simulink model "NBMS_App_Harness1"  (R2026b)
settings: Solver=FixedStepDiscrete  StopTime=25  FixedStep=0.1
undefined symbols (not defined in the file): Active_DisChrg_E, BMS_BattSoCDerate_E, BMS_BattTempDerate_E, BMS_DCDCMosfet_STS_E, BMS_HVMosfet_STS_E, BMS_MODE_E, BMS_NM_Msg_E, BMS_PMosfet_STS_E, Charger_Mode_E, Charger_Mode_Req_E, CV_Mode_Timer_E, OBC_E, VDU_MACHINE_STS_E
(part 1 of 4)
settings Model: PauseTimes=12  Creator=rathi  LastModifiedBy=rathi
settings OptimizationCC: DefaultParameterBehavior=Inlined  DifferentSizesBufferReuse=on  EfficientTunableParamExpr=on  EnhancedBackFolding=on  OptimizationCustomize=off  OptimizeBlockOrder=speed  PassReuseOutputArgsAs=Individual arguments  RemoveInternalMemoryZeroInit=on  RemoveRootLevelIOMemoryZeroInit=on
settings DebuggingCC: ParameterTunabilityLossMsg=error
settings SFSimCC: MATLABDynamicMemAlloc=off
settings RTWCC: Description=Embedded Coder  GenCodeOnly=on  PackageGeneratedCodeAndArtifacts=on  SystemTargetFile=ert.tlc  TemplateMakefile=ert_default_tmf
settings CodeAppCC: ForceParamTrailComments=on  IgnoreCustomStorageClasses=off  InsertBlockDesc=on  OperatorAnnotations=on  SFDataObjDesc=on  SimulinkDataObjDesc=on
settings ERTTargetCC: DynamicArrayContainerType=coder::array  GenerateSampleERTMain=on
settings ConfigComp: DVDefectChecker=on  DVDetectOutOfBounds=on  DVHarnessSource=Signal Editor  DVModelReferenceHarness=on  DVTestSuiteOptimization=Auto

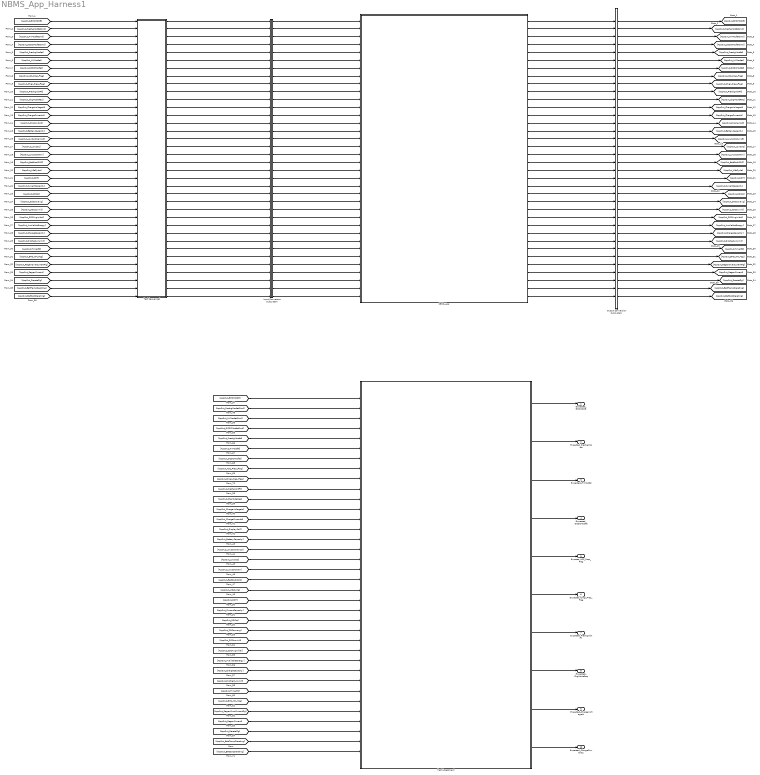
== system NBMS_App_Harness1 ==
  Input Conversion Subsystem : Subsystem  Tag=__SLT_ICS__  Description=|
      | Signal spec.
      | and routing
      settings: AttributesFormatString=%<Description>
  NBMS_App : ModelReference  ModelNameDialog=NBMS_App  SimulationMode=Normal  ModelReferenceVersion=1.0
  Output Conversion Subsystem : Subsystem  Tag=__SLT_OCS__  Description=|
      | Signal spec.
      | and routing
      settings: AttributesFormatString=%<Description>
  Test Assessment : Test Sequence  TreatAsAtomicUnit=on
  Test Sequence1 : Test Sequence  TreatAsAtomicUnit=on
  Expected_BMSMODE : Outport
  Expected_PrechgMosfet : Outport  Port=2
  Expected_HVMosfet : Outport  Port=3
  Expected_DCDCMosfet : Outport  Port=4
  Expcted_ASC_Prep_Flag : Outport  Port=5
  Expected_Chrgr_Prep_Flag : Outport  Port=6
  Expected_PrechgVoltFlt : Outport  Port=7
  Expected_ChgModeReq : Outport  Port=8
  Expected_ChargeVoltageLt : Outport  Port=9
  Expected_ChargeCurrentLt : Outport  Port=10
  wires:
  Test Sequence1/1(AppIn_HardwiredIgn) -> Input Conversion Subsystem/1(Inport_1)
  Test Sequence1/2(AppIn_OBCwakeup) -> Input Conversion Subsystem/2(Inport_2)
  Test Sequence1/3(AppIn_RTCwakeup) -> Input Conversion Subsystem/3(Inport_3)
  Test Sequence1/4(AppIn_MCUHVIL) -> Input Conversion Subsystem/4(Inport_4)
  Test Sequence1/5(AppIn_OBCHVIL) -> Input Conversion Subsystem/5(Inport_5)
  Test Sequence1/6(AppIn_SoCLEDSW) -> Input Conversion Subsystem/6(Inport_6)
  Test Sequence1/7(AppIn_ChgMode) -> Input Conversion Subsystem/7(Inport_7)
  Test Sequence1/8(AppIn_CVmodeTimer) -> Input Conversion Subsystem/8(Inport_8)
  Test Sequence1/9(AppIn_TRerror) -> Input Conversion Subsystem/9(Inport_9)
  Test Sequence1/10(AppIn_TRtimer) -> Input Conversion Subsystem/10(Inport_10)
  Test Sequence1/11(AppIn_G3CommonFlt) -> Input Conversion Subsystem/11(Inport_11)
  Test Sequence1/12(AppIn_G3DischargeFlt) -> Input Conversion Subsystem/12(Inport_12)
  Test Sequence1/13(AppIn_G4T1DischargeFlt) -> Input Conversion Subsystem/13(Inport_13)
  Test Sequence1/14(AppIn_G4T2DischargeFlt) -> Input Conversion Subsystem/14(Inport_14)
  Test Sequence1/15(AppIn_G4CommonFlt) -> Input Conversion Subsystem/15(Inport_15)
  Test Sequence1/16(AppIn_G4ChargeFlt) -> Input Conversion Subsystem/16(Inport_16)
  Test Sequence1/17(AppIn_OBCHeartbeatFail) -> Input Conversion Subsystem/17(Inport_17)
  Test Sequence1/18(AppIn_LoadVolt) -> Input Conversion Subsystem/18(Inport_18)
  Test Sequence1/19(AppIn_PackVolt) -> Input Conversion Subsystem/19(Inport_19)
  Test Sequence1/20(AppIn_ActiveDischg) -> Input Conversion Subsystem/20(Inport_20)
  Test Sequence1/21(AppIn_BattTemp) -> Input Conversion Subsystem/21(Inport_21)
  Test Sequence1/22(AppIn_BattCurrent) -> Input Conversion Subsystem/22(Inport_22)
  Test Sequence1/23(AppIn_BattVoltages) -> Input Conversion Subsystem/23(Inport_23)
  Test Sequence1/24(AppIn_LastStoredSOC) -> Input Conversion Subsystem/24(Inport_24)
  Test Sequence1/25(AppIn_LastStoredCycle) -> Input Conversion Subsystem/25(Inport_25)
  Test Sequence1/26(AppIn_I2Cerror) -> Input Conversion Subsystem/26(Inport_26)
  Test Sequence1/27(AppIn_LastStoredSOH) -> Input Conversion Subsystem/27(Inport_27)
  Test Sequence1/28(AppIn_MachineStatus) -> Input Conversion Subsystem/28(Inport_28)
  Test Sequence1/29(AppIn_HVMosfetfb) -> Input Conversion Subsystem/29(Inport_29)
  Test Sequence1/30(AppIn_DCDCMosfetfb) -> Input Conversion Subsystem/30(Inport_30)
  Test Sequence1/31(AppIn_PMosfetfb) -> Input Conversion Subsystem/31(Inport_31)
  Test Sequence1/32(AppIn_BMSVltSnsrFail) -> Input Conversion Subsystem/32(Inport_32)
  Test Sequence1/33(AppIn_BattPackTempSnsrFail) -> Input Conversion Subsystem/33(Inport_33)
  Test Sequence1/34(AppIn_VltImbFlt) -> Input Conversion Subsystem/34(Inport_34)
  Test Sequence1/35(AppIn_TempImbWarn) -> Input Conversion Subsystem/35(Inport_35)
  Test Sequence1/36(AppIn_EEPROMSoCWarn15) -> Input Conversion Subsystem/36(Inport_36)
  [AppOut_BMSMODE] -> Test Sequence1/1(AppOut_BMSMODE)
  [AppOut_PrechgMosfetCmd] -> Test Sequence1/2(AppOut_PrechgMosfetCmd)
  [AppOut_HVMosfetCmd] -> Test Sequence1/3(AppOut_HVMosfetCmd)
  [AppOut_DCDCMosfetCmd] -> Test Sequence1/4(AppOut_DCDCMosfetCmd)
  [AppOut_PrechgMosfet] -> Test Sequence1/5(AppOut_PrechgMosfet)
  [AppOut_HVMosfet] -> Test Sequence1/6(AppOut_HVMosfet)
  [AppOut_DCDCMosfet] -> Test Sequence1/7(AppOut_DCDCMosfet)
  [AppOut_ASC_Prep_Flag] -> Test Sequence1/8(AppOut_ASC_Prep_Flag)
  [AppOut_Chrgr_Prep_Flag] -> Test Sequence1/9(AppOut_Chrgr_Prep_Flag)
  [AppOut_PrechgVoltFlt] -> Test Sequence1/10(AppOut_PrechgVoltFlt)
  [AppOut_ChgModeReq] -> Test Sequence1/11(AppOut_ChgModeReq)
  [AppOut_ChargeVoltageLt] -> Test Sequence1/12(AppOut_ChargeVoltageLt)
  [AppOut_ChargeCurrentLt] -> Test Sequence1/13(AppOut_ChargeCurrentLt)
  [AppOut_DisplaySoC] -> Test Sequence1/14(AppOut_DisplaySoC)
  [AppOut_BatteryCapacity] -> Test Sequence1/15(AppOut_BatteryCapacity)
  [AppOut_LowSoCWarn15] -> Test Sequence1/16(AppOut_LowSoCWarn15)
  [AppOut_LowSoC] -> Test Sequence1/17(AppOut_LowSoC)
  [AppOut_LowSoCWarn] -> Test Sequence1/18(AppOut_LowSoCWarn)
  [AppOut_BattPackSOC] -> Test Sequence1/19(AppOut_BattPackSOC)
  [AppOut_LifeCycle] -> Test Sequence1/20(AppOut_LifeCycle)
  [AppOut_SOH] -> Test Sequence1/21(AppOut_SOH)
  [AppOut_CurrentCapacity] -> Test Sequence1/22(AppOut_CurrentCapacity)
  [AppOut_SOCcc] -> Test Sequence1/23(AppOut_SOCcc)
  [AppOut_SOCocvavg] -> Test Sequence1/24(AppOut_SOCocvavg)
  [AppOut_SOCocvInit] -> Test Sequence1/25(AppOut_SOCocvInit)
  [AppOut_SOCAvgInitial] -> Test Sequence1/26(AppOut_SOCAvgInitial)
  [AppOut_AvailableEnergy] -> Test Sequence1/27(AppOut_AvailableEnergy)
  [AppOut_ChargeCapacity] -> Test Sequence1/28(AppOut_ChargeCapacity)
  [AppOut_DischgCurrLimit] -> Test Sequence1/29(AppOut_DischgCurrLimit)
  [AppOut_Timer30] -> Test Sequence1/30(AppOut_Timer30)
  [AppOut_BMS_NM_Msg] -> Test Sequence1/31(AppOut_BMS_NM_Msg)
  [AppOut_RegenOverCurrentFlg] -> Test Sequence1/32(AppOut_RegenOverCurrentFlg)
  [AppOut_RegenCurrent] -> Test Sequence1/33(AppOut_RegenCurrent)
  [AppOut_DerateFlg] -> Test Sequence1/34(AppOut_DerateFlg)
  [AppOut_BattTempDerating] -> Test Sequence1/35(AppOut_BattTempDerating)
  [AppOut_BattSoCDerating] -> Test Sequence1/36(AppOut_BattSoCDerating)
  Output Conversion Subsystem/1(Outport_1) -> [AppOut_BMSMODE]  "AppOut_BMSMODE"
  Output Conversion Subsystem/2(Outport_2) -> [AppOut_PrechgMosfetCmd]  "AppOut_PrechgMosfetCmd"
  Output Conversion Subsystem/3(Outport_3) -> [AppOut_HVMosfetCmd]  "AppOut_HVMosfetCmd"
  Output Conversion Subsystem/4(Outport_4) -> [AppOut_DCDCMosfetCmd]  "AppOut_DCDCMosfetCmd"
  Output Conversion Subsystem/5(Outport_5) -> [AppOut_PrechgMosfet]  "AppOut_PrechgMosfet"
  Output Conversion Subsystem/6(Outport_6) -> [AppOut_HVMosfet]  "AppOut_HVMosfet"
  Output Conversion Subsystem/7(Outport_7) -> [AppOut_DCDCMosfet]  "AppOut_DCDCMosfet"
  Output Conversion Subsystem/8(Outport_8) -> [AppOut_ASC_Prep_Flag]  "AppOut_ASC_Prep_Flag"
  Output Conversion Subsystem/9(Outport_9) -> [AppOut_Chrgr_Prep_Flag]  "AppOut_Chrgr_Prep_Flag"
  Output Conversion Subsystem/10(Outport_10) -> [AppOut_PrechgVoltFlt]  "AppOut_PrechgVoltFlt"
  Output Conversion Subsystem/11(Outport_11) -> [AppOut_ChgModeReq]  "AppOut_ChgModeReq"
  Output Conversion Subsystem/12(Outport_12) -> [AppOut_ChargeVoltageLt]  "AppOut_ChargeVoltageLt"
  Output Conversion Subsystem/13(Outport_13) -> [AppOut_ChargeCurrentLt]  "AppOut_ChargeCurrentLt"
  Output Conversion Subsystem/14(Outport_14) -> [AppOut_DisplaySoC]  "AppOut_DisplaySoC"
  Output Conversion Subsystem/15(Outport_15) -> [AppOut_BatteryCapacity]  "AppOut_BatteryCapacity"
  Output Conversion Subsystem/16(Outport_16) -> [AppOut_LowSoCWarn15]  "AppOut_LowSoCWarn15"
  Output Conversion Subsystem/17(Outport_17) -> [AppOut_LowSoC]  "AppOut_LowSoC"
  Output Conversion Subsystem/18(Outport_18) -> [AppOut_LowSoCWarn]  "AppOut_LowSoCWarn"
  Output Conversion Subsystem/19(Outport_19) -> [AppOut_BattPackSOC]  "AppOut_BattPackSOC"
  Output Conversion Subsystem/20(Outport_20) -> [AppOut_LifeCycle]  "AppOut_LifeCycle"
  Output Conversion Subsystem/21(Outport_21) -> [AppOut_SOH]  "AppOut_SOH"
  Output Conversion Subsystem/22(Outport_22) -> [AppOut_CurrentCapacity]  "AppOut_CurrentCapacity"
  Output Conversion Subsystem/23(Outport_23) -> [AppOut_SOCcc]  "AppOut_SOCcc"
  Output Conversion Subsystem/24(Outport_24) -> [AppOut_SOCocvavg]  "AppOut_SOCocvavg"
  Output Conversion Subsystem/25(Outport_25) -> [AppOut_SOCocvInit]  "AppOut_SOCocvInit"
  Output Conversion Subsystem/26(Outport_26) -> [AppOut_SOCAvgInitial]  "AppOut_SOCAvgInitial"
  Output Conversion Subsystem/27(Outport_27) -> [AppOut_AvailableEnergy]  "AppOut_AvailableEnergy"
  Output Conversion Subsystem/28(Outport_28) -> [AppOut_ChargeCapacity]  "AppOut_ChargeCapacity"
  Output Conversion Subsystem/29(Outport_29) -> [AppOut_DischgCurrLimit]  "AppOut_DischgCurrLimit"
  Output Conversion Subsystem/30(Outport_30) -> [AppOut_Timer30]  "AppOut_Timer30"
  Output Conversion Subsystem/31(Outport_31) -> [AppOut_BMS_NM_Msg]  "AppOut_BMS_NM_Msg"
  Output Conversion Subsystem/32(Outport_32) -> [AppOut_RegenOverCurrentFlg]  "AppOut_RegenOverCurrentFlg"
  Output Conversion Subsystem/33(Outport_33) -> [AppOut_RegenCurrent]  "AppOut_RegenCurrent"
  Output Conversion Subsystem/34(Outport_34) -> [AppOut_DerateFlg]  "AppOut_DerateFlg"
  Output Conversion Subsystem/35(Outport_35) -> [AppOut_BattTempDerating]  "AppOut_BattTempDerating"
  Output Conversion Subsystem/36(Outport_36) -> [AppOut_BattSoCDerating]  "AppOut_BattSoCDerating"
  [AppOut_Chrgr_Prep_Flag] -> Test Assessment/9(AppOut_Chrgr_Prep_Flag)
  [AppOut_BattSoCDerating] -> Test Assessment/36(AppOut_BattSoCDerating)
  Test Assessment/1(Expected_BMSMODE) -> Expected_BMSMODE/1
  [AppOut_PrechgMosfet] -> Test Assessment/5(AppOut_PrechgMosfet)
  [AppOut_ChargeCapacity] -> Test Assessment/28(AppOut_ChargeCapacity)
  [AppOut_DerateFlg] -> Test Assessment/34(AppOut_DerateFlg)
  [AppOut_BMSMODE] -> Test Assessment/1(AppOut_BMSMODE)
  [AppOut_LowSoCWarn15] -> Test Assessment/16(AppOut_LowSoCWarn15)
  [AppOut_SOCocvInit] -> Test Assessment/25(AppOut_SOCocvInit)
  [AppOut_HVMosfet] -> Test Assessment/6(AppOut_HVMosfet)
  [AppOut_DisplaySoC] -> Test Assessment/14(AppOut_DisplaySoC)
  [AppOut_DischgCurrLimit] -> Test Assessment/29(AppOut_DischgCurrLimit)
  [AppOut_Timer30] -> Test Assessment/30(AppOut_Timer30)
  Test Assessment/4(Expected_DCDCMosfet) -> Expected_DCDCMosfet/1
  [AppOut_BatteryCapacity] -> Test Assessment/15(AppOut_BatteryCapacity)
  Test Assessment/7(Expected_PrechgVoltFlt) -> Expected_PrechgVoltFlt/1
  [AppOut_BMS_NM_Msg] -> Test Assessment/31(AppOut_BMS_NM_Msg)
  [AppOut_SOCAvgInitial] -> Test Assessment/26(AppOut_SOCAvgInitial)
  [AppOut_RegenOverCurrentFlg] -> Test Assessment/32(AppOut_RegenOverCurrentFlg)
  Test Assessment/6(Expected_Chrgr_Prep_Flag) -> Expected_Chrgr_Prep_Flag/1
  [AppOut_LifeCycle] -> Test Assessment/20(AppOut_LifeCycle)
  [AppOut_RegenCurrent] -> Test Assessment/33(AppOut_RegenCurrent)
  [AppOut_HVMosfetCmd] -> Test Assessment/3(AppOut_HVMosfetCmd)
  [AppOut_PrechgMosfetCmd] -> Test Assessment/2(AppOut_PrechgMosfetCmd)
  [AppOut_BattTempDerating] -> Test Assessment/35(AppOut_BattTempDerating)
  [AppOut_PrechgVoltFlt] -> Test Assessment/10(AppOut_PrechgVoltFlt)
  [AppOut_SOH] -> Test Assessment/21(AppOut_SOH)
  [AppOut_ChargeVoltageLt] -> Test Assessment/12(AppOut_ChargeVoltageLt)
  [AppOut_LowSoCWarn] -> Test Assessment/18(AppOut_LowSoCWarn)
  Test Assessment/3(Expected_HVMosfet) -> Expected_HVMosfet/1
  [AppOut_ASC_Prep_Flag] -> Test Assessment/8(AppOut_ASC_Prep_Flag)
  [AppOut_CurrentCapacity] -> Test Assessment/22(AppOut_CurrentCapacity)
  [AppOut_AvailableEnergy] -> Test Assessment/27(AppOut_AvailableEnergy)
  Test Assessment/5(Expected_ASC_Prep_Flag) -> Expcted_ASC_Prep_Flag/1
  [AppOut_ChgModeReq] -> Test Assessment/11(AppOut_ChgModeReq)
  [AppOut_SOCcc] -> Test Assessment/23(AppOut_SOCcc)
  Test Assessment/2(Expected_PrechgMosfet) -> Expected_PrechgMosfet/1
  [AppOut_BattPackSOC] -> Test Assessment/19(AppOut_BattPackSOC)
  [AppOut_DCDCMosfet] -> Test Assessment/7(AppOut_DCDCMosfet)
  [AppOut_LowSoC] -> Test Assessment/17(AppOut_LowSoC)
  [AppOut_DCDCMosfetCmd] -> Test Assessment/4(AppOut_DCDCMosfetCmd)
  [AppOut_SOCocvavg] -> Test Assessment/24(AppOut_SOCocvavg)
  [AppOut_ChargeCurrentLt] -> Test Assessment/13(AppOut_ChargeCurrentLt)
  Test Assessment/8(Expected_ChgModeReq) -> Expected_ChgModeReq/1
  Test Assessment/9(Expected_ChargeVoltageLt) -> Expected_ChargeVoltageLt/1
  Test Assessment/10(Expected_ChargeCurrentLt) -> Expected_ChargeCurrentLt/1
  NBMS_App/1 -> Output Conversion Subsystem/1(Inport_1)
  NBMS_App/2 -> Output Conversion Subsystem/2(Inport_2)
  NBMS_App/3 -> Output Conversion Subsystem/3(Inport_3)
  NBMS_App/4 -> Output Conversion Subsystem/4(Inport_4)
  NBMS_App/5 -> Output Conversion Subsystem/5(Inport_5)
  NBMS_App/6 -> Output Conversion Subsystem/6(Inport_6)
  NBMS_App/7 -> Output Conversion Subsystem/7(Inport_7)
  NBMS_App/8 -> Output Conversion Subsystem/8(Inport_8)
  NBMS_App/9 -> Output Conversion Subsystem/9(Inport_9)
  NBMS_App/10 -> Output Conversion Subsystem/10(Inport_10)
  NBMS_App/11 -> Output Conversion Subsystem/11(Inport_11)
  NBMS_App/12 -> Output Conversion Subsystem/12(Inport_12)
  NBMS_App/13 -> Output Conversion Subsystem/13(Inport_13)
  NBMS_App/14 -> Output Conversion Subsystem/14(Inport_14)
  NBMS_App/15 -> Output Conversion Subsystem/15(Inport_15)
  NBMS_App/16 -> Output Conversion Subsystem/16(Inport_16)
  NBMS_App/17 -> Output Conversion Subsystem/17(Inport_17)
  NBMS_App/18 -> Output Conversion Subsystem/18(Inport_18)
  NBMS_App/19 -> Output Conversion Subsystem/19(Inport_19)
  NBMS_App/20 -> Output Conversion Subsystem/20(Inport_20)
  NBMS_App/21 -> Output Conversion Subsystem/21(Inport_21)
  NBMS_App/22 -> Output Conversion Subsystem/22(Inport_22)
  NBMS_App/23 -> Output Conversion Subsystem/23(Inport_23)
  NBMS_App/24 -> Output Conversion Subsystem/24(Inport_24)
  NBMS_App/25 -> Output Conversion Subsystem/25(Inport_25)
  NBMS_App/26 -> Output Conversion Subsystem/26(Inport_26)
  NBMS_App/27 -> Output Conversion Subsystem/27(Inport_27)
  NBMS_App/28 -> Output Conversion Subsystem/28(Inport_28)
  NBMS_App/29 -> Output Conversion Subsystem/29(Inport_29)
  NBMS_App/30 -> Output Conversion Subsystem/30(Inport_30)
  NBMS_App/31 -> Output Conversion Subsystem/31(Inport_31)
  NBMS_App/32 -> Output Conversion Subsystem/32(Inport_32)
  NBMS_App/33 -> Output Conversion Subsystem/33(Inport_33)
  NBMS_App/34 -> Output Conversion Subsystem/34(Inport_34)
  NBMS_App/35 -> Output Conversion Subsystem/35(Inport_35)
  NBMS_App/36 -> Output Conversion Subsystem/36(Inport_36)
  Input Conversion Subsystem/1(Outport_1) -> NBMS_App/1  "AppIn_HardwiredIgn"
  Input Conversion Subsystem/2(Outport_2) -> NBMS_App/2  "AppIn_OBCwakeup"
  Input Conversion Subsystem/3(Outport_3) -> NBMS_App/3  "AppIn_RTCwakeup"
  Input Conversion Subsystem/4(Outport_4) -> NBMS_App/4  "AppIn_MCUHVIL"
  Input Conversion Subsystem/5(Outport_5) -> NBMS_App/5  "AppIn_OBCHVIL"
  Input Conversion Subsystem/6(Outport_6) -> NBMS_App/6  "AppIn_SoCLEDSW"
  Input Conversion Subsystem/7(Outport_7) -> NBMS_App/7  "AppIn_ChgMode"
  Input Conversion Subsystem/8(Outport_8) -> NBMS_App/8  "AppIn_CVmodeTimer"
  Input Conversion Subsystem/9(Outport_9) -> NBMS_App/9  "AppIn_TRerror"
  Input Conversion Subsystem/10(Outport_10) -> NBMS_App/10  "AppIn_TRtimer"
  Input Conversion Subsystem/11(Outport_11) -> NBMS_App/11  "AppIn_G3CommonFlt"
  Input Conversion Subsystem/12(Outport_12) -> NBMS_App/12  "AppIn_G3DischargeFlt"
  Input Conversion Subsystem/13(Outport_13) -> NBMS_App/13  "AppIn_G4T1DischargeFlt"
  Input Conversion Subsystem/14(Outport_14) -> NBMS_App/14  "AppIn_G4T2DischargeFlt"
  Input Conversion Subsystem/15(Outport_15) -> NBMS_App/15  "AppIn_G4CommonFlt"
  Input Conversion Subsystem/16(Outport_16) -> NBMS_App/16  "AppIn_G4ChargeFlt"
  Input Conversion Subsystem/17(Outport_17) -> NBMS_App/17  "AppIn_OBCHeartbeatFail"
  Input Conversion Subsystem/18(Outport_18) -> NBMS_App/18  "AppIn_LoadVolt"
  Input Conversion Subsystem/19(Outport_19) -> NBMS_App/19  "AppIn_PackVolt"
  Input Conversion Subsystem/20(Outport_20) -> NBMS_App/20  "AppIn_ActiveDischg"
  Input Conversion Subsystem/21(Outport_21) -> NBMS_App/21  "AppIn_BattTemp"
  Input Conversion Subsystem/22(Outport_22) -> NBMS_App/22  "AppIn_BattCurrent"
  Input Conversion Subsystem/23(Outport_23) -> NBMS_App/23  "AppIn_BattVoltages"
  Input Conversion Subsystem/24(Outport_24) -> NBMS_App/24  "AppIn_LastStoredSOC"
  Input Conversion Subsystem/25(Outport_25) -> NBMS_App/25  "AppIn_LastStoredCycle"
  Input Conversion Subsystem/26(Outport_26) -> NBMS_App/26  "AppIn_I2Cerror"
  Input Conversion Subsystem/27(Outport_27) -> NBMS_App/27  "AppIn_LastStoredSOH"
  Input Conversion Subsystem/28(Outport_28) -> NBMS_App/28  "AppIn_MachineStatus"
  Input Conversion Subsystem/29(Outport_29) -> NBMS_App/29  "AppIn_HVMosfetfb"
  Input Conversion Subsystem/30(Outport_30) -> NBMS_App/30  "AppIn_DCDCMosfetfb"
  Input Conversion Subsystem/31(Outport_31) -> NBMS_App/31  "AppIn_PMosfetfb"
  Input Conversion Subsystem/32(Outport_32) -> NBMS_App/32  "AppIn_BMSVltSnsrFail"
  Input Conversion Subsystem/33(Outport_33) -> NBMS_App/33  "AppIn_BattPackTempSnsrFail"
  Input Conversion Subsystem/34(Outport_34) -> NBMS_App/34  "AppIn_VltImbFlt"
  Input Conversion Subsystem/35(Outport_35) -> NBMS_App/35  "AppIn_TempImbWarn"
  Input Conversion Subsystem/36(Outport_36) -> NBMS_App/36  "AppIn_EEPROMSoCWarn15"

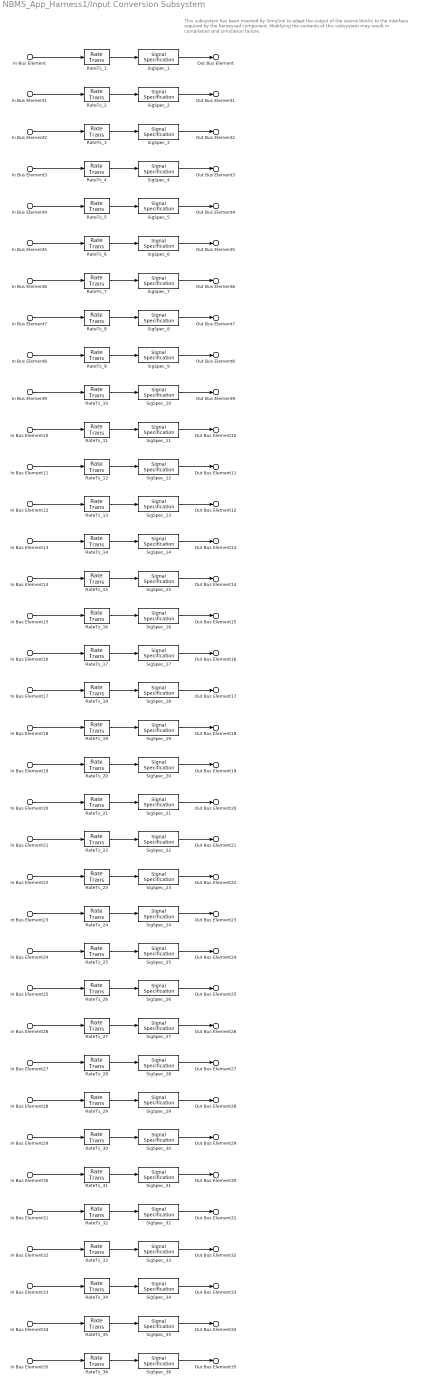
== system NBMS_App_Harness1/Input Conversion Subsystem ==
  note: This subsystem has been inserted by Simulink to adapt the output of the source blocks to the interface required by the harnessed component.
      |  Modifying the contents of this subsystem may result in compilation and simulation failure.
  In Bus Element : Inport  PortName=Inport_1
  In Bus Element1 : Inport  Port=2  PortName=Inport_2
  In Bus Element2 : Inport  Port=3  PortName=Inport_3
  In Bus Element3 : Inport  Port=4  PortName=Inport_4
  In Bus Element4 : Inport  Port=5  PortName=Inport_5
  In Bus Element5 : Inport  Port=6  PortName=Inport_6
  In Bus Element6 : Inport  Port=7  PortName=Inport_7
  In Bus Element7 : Inport  Port=8  PortName=Inport_8
  In Bus Element8 : Inport  Port=9  PortName=Inport_9
  In Bus Element9 : Inport  Port=10  PortName=Inport_10
  In Bus Element10 : Inport  Port=11  PortName=Inport_11
  In Bus Element11 : Inport  Port=12  PortName=Inport_12
  In Bus Element12 : Inport  Port=13  PortName=Inport_13
  In Bus Element13 : Inport  Port=14  PortName=Inport_14
  In Bus Element14 : Inport  Port=15  PortName=Inport_15
  In Bus Element15 : Inport  Port=16  PortName=Inport_16
  In Bus Element16 : Inport  Port=17  PortName=Inport_17
  In Bus Element17 : Inport  Port=18  PortName=Inport_18
  In Bus Element18 : Inport  Port=19  PortName=Inport_19
  In Bus Element19 : Inport  Port=20  PortName=Inport_20
  In Bus Element20 : Inport  Port=21  PortName=Inport_21
  In Bus Element21 : Inport  Port=22  PortName=Inport_22
  In Bus Element22 : Inport  Port=23  PortName=Inport_23
  In Bus Element23 : Inport  Port=24  PortName=Inport_24
  In Bus Element24 : Inport  Port=25  PortName=Inport_25
  In Bus Element25 : Inport  Port=26  PortName=Inport_26
  In Bus Element26 : Inport  Port=27  PortName=Inport_27
  In Bus Element27 : Inport  Port=28  PortName=Inport_28
  In Bus Element28 : Inport  Port=29  PortName=Inport_29
  In Bus Element29 : Inport  Port=30  PortName=Inport_30
  In Bus Element30 : Inport  Port=31  PortName=Inport_31
  In Bus Element31 : Inport  Port=32  PortName=Inport_32
  In Bus Element32 : Inport  Port=33  PortName=Inport_33
  In Bus Element33 : Inport  Port=34  PortName=Inport_34
  In Bus Element34 : Inport  Port=35  PortName=Inport_35
  In Bus Element35 : Inport  Port=36  PortName=Inport_36
  RateTs_{1,3..6,9..19,21..27,29..36} (31 alike) : RateTransition  OutPortSampleTime=0.1
  RateTs_2 : RateTransition  InitialCondition=OBC_E.Sleep  OutPortSampleTime=0.1
  RateTs_20 : RateTransition  InitialCondition=Active_DisChrg_E.Inactive  OutPortSampleTime=0.1
  RateTs_28 : RateTransition  InitialCondition=VDU_MACHINE_STS_E.SNA  OutPortSampleTime=0.1
  RateTs_7 : RateTransition  InitialCondition=Charger_Mode_E.OFF  OutPortSampleTime=0.1
  RateTs_8 : RateTransition  InitialCondition=CV_Mode_Timer_E.Off  OutPortSampleTime=0.1
  SigSpec_{1,3..6,9..17,26,29..36} (23 alike) : SignalSpecification  OutDataTypeStr=boolean  Dimensions=[1]  SampleTime=0.1
  SigSpec_{18..19,22,24..25,27} (6 alike) : SignalSpecification  OutDataTypeStr=double  Dimensions=[1]  SampleTime=0.1
  SigSpec_2 : SignalSpecification  OutDataTypeStr=Enum: OBC_E  Dimensions=[1]  SampleTime=0.1
  SigSpec_20 : SignalSpecification  OutDataTypeStr=Enum: Active_DisChrg_E  Dimensions=[1]  SampleTime=0.1
  SigSpec_21 : SignalSpecification  OutDataTypeStr=double  Dimensions=[6, 1]  SampleTime=0.1
  SigSpec_23 : SignalSpecification  OutDataTypeStr=double  Dimensions=[20, 1]  SampleTime=0.1
  SigSpec_28 : SignalSpecification  OutDataTypeStr=Enum: VDU_MACHINE_STS_E  Dimensions=[1]  SampleTime=0.1
  SigSpec_7 : SignalSpecification  OutDataTypeStr=Enum: Charger_Mode_E  Dimensions=[1]  SampleTime=0.1
  SigSpec_8 : SignalSpecification  OutDataTypeStr=Enum: CV_Mode_Timer_E  Dimensions=[1]  SampleTime=0.1
  Out Bus Element : Outport  PortName=Outport_1
  Out Bus Element1 : Outport  Port=2  PortName=Outport_2
  Out Bus Element2 : Outport  Port=3  PortName=Outport_3
  Out Bus Element3 : Outport  Port=4  PortName=Outport_4
  Out Bus Element4 : Outport  Port=5  PortName=Outport_5
  Out Bus Element5 : Outport  Port=6  PortName=Outport_6
  Out Bus Element6 : Outport  Port=7  PortName=Outport_7
  Out Bus Element7 : Outport  Port=8  PortName=Outport_8
  Out Bus Element8 : Outport  Port=9  PortName=Outport_9
  Out Bus Element9 : Outport  Port=10  PortName=Outport_10
  Out Bus Element10 : Outport  Port=11  PortName=Outport_11
  Out Bus Element11 : Outport  Port=12  PortName=Outport_12
  Out Bus Element12 : Outport  Port=13  PortName=Outport_13
  Out Bus Element13 : Outport  Port=14  PortName=Outport_14
  Out Bus Element14 : Outport  Port=15  PortName=Outport_15
  Out Bus Element15 : Outport  Port=16  PortName=Outport_16
  Out Bus Element16 : Outport  Port=17  PortName=Outport_17
  Out Bus Element17 : Outport  Port=18  PortName=Outport_18
  Out Bus Element18 : Outport  Port=19  PortName=Outport_19
  Out Bus Element19 : Outport  Port=20  PortName=Outport_20
  Out Bus Element20 : Outport  Port=21  PortName=Outport_21
  Out Bus Element21 : Outport  Port=22  PortName=Outport_22
  Out Bus Element22 : Outport  Port=23  PortName=Outport_23
  Out Bus Element23 : Outport  Port=24  PortName=Outport_24
  Out Bus Element24 : Outport  Port=25  PortName=Outport_25
  Out Bus Element25 : Outport  Port=26  PortName=Outport_26
  Out Bus Element26 : Outport  Port=27  PortName=Outport_27
  Out Bus Element27 : Outport  Port=28  PortName=Outport_28
  Out Bus Element28 : Outport  Port=29  PortName=Outport_29
  Out Bus Element29 : Outport  Port=30  PortName=Outport_30
  Out Bus Element30 : Outport  Port=31  PortName=Outport_31
  Out Bus Element31 : Outport  Port=32  PortName=Outport_32
  Out Bus Element32 : Outport  Port=33  PortName=Outport_33
  Out Bus Element33 : Outport  Port=34  PortName=Outport_34
  Out Bus Element34 : Outport  Port=35  PortName=Outport_35
  Out Bus Element35 : Outport  Port=36  PortName=Outport_36
  wires:
  SigSpec_1/1 -> Out Bus Element/1
  RateTs_1/1 -> SigSpec_1/1
  In Bus Element/1 -> RateTs_1/1
  SigSpec_2/1 -> Out Bus Element1/1
  RateTs_2/1 -> SigSpec_2/1
  In Bus Element1/1 -> RateTs_2/1
  SigSpec_3/1 -> Out Bus Element2/1
  RateTs_3/1 -> SigSpec_3/1
  In Bus Element2/1 -> RateTs_3/1
  SigSpec_4/1 -> Out Bus Element3/1
  RateTs_4/1 -> SigSpec_4/1
  In Bus Element3/1 -> RateTs_4/1
  SigSpec_5/1 -> Out Bus Element4/1
  RateTs_5/1 -> SigSpec_5/1
  In Bus Element4/1 -> RateTs_5/1
  SigSpec_6/1 -> Out Bus Element5/1
  RateTs_6/1 -> SigSpec_6/1
  In Bus Element5/1 -> RateTs_6/1
  SigSpec_7/1 -> Out Bus Element6/1
  RateTs_7/1 -> SigSpec_7/1
  In Bus Element6/1 -> RateTs_7/1
  SigSpec_8/1 -> Out Bus Element7/1
  RateTs_8/1 -> SigSpec_8/1
  In Bus Element7/1 -> RateTs_8/1
  SigSpec_9/1 -> Out Bus Element8/1
  RateTs_9/1 -> SigSpec_9/1
  In Bus Element8/1 -> RateTs_9/1
  SigSpec_10/1 -> Out Bus Element9/1
  RateTs_10/1 -> SigSpec_10/1
  In Bus Element9/1 -> RateTs_10/1
  SigSpec_11/1 -> Out Bus Element10/1
  RateTs_11/1 -> SigSpec_11/1
  In Bus Element10/1 -> RateTs_11/1
  SigSpec_12/1 -> Out Bus Element11/1
  RateTs_12/1 -> SigSpec_12/1
  In Bus Element11/1 -> RateTs_12/1
  SigSpec_13/1 -> Out Bus Element12/1
  RateTs_13/1 -> SigSpec_13/1
  In Bus Element12/1 -> RateTs_13/1
  SigSpec_14/1 -> Out Bus Element13/1
  RateTs_14/1 -> SigSpec_14/1
  In Bus Element13/1 -> RateTs_14/1
  SigSpec_15/1 -> Out Bus Element14/1
  RateTs_15/1 -> SigSpec_15/1
  In Bus Element14/1 -> RateTs_15/1
  SigSpec_16/1 -> Out Bus Element15/1
  RateTs_16/1 -> SigSpec_16/1
  In Bus Element15/1 -> RateTs_16/1
  SigSpec_17/1 -> Out Bus Element16/1
  RateTs_17/1 -> SigSpec_17/1
  In Bus Element16/1 -> RateTs_17/1
  SigSpec_18/1 -> Out Bus Element17/1
  RateTs_18/1 -> SigSpec_18/1
  In Bus Element17/1 -> RateTs_18/1
  SigSpec_19/1 -> Out Bus Element18/1
  RateTs_19/1 -> SigSpec_19/1
  In Bus Element18/1 -> RateTs_19/1
  SigSpec_20/1 -> Out Bus Element19/1
  RateTs_20/1 -> SigSpec_20/1
  In Bus Element19/1 -> RateTs_20/1
  SigSpec_21/1 -> Out Bus Element20/1
  RateTs_21/1 -> SigSpec_21/1
  In Bus Element20/1 -> RateTs_21/1
  SigSpec_22/1 -> Out Bus Element21/1
  RateTs_22/1 -> SigSpec_22/1
  In Bus Element21/1 -> RateTs_22/1
  SigSpec_23/1 -> Out Bus Element22/1
  RateTs_23/1 -> SigSpec_23/1
  In Bus Element22/1 -> RateTs_23/1
  SigSpec_24/1 -> Out Bus Element23/1
  RateTs_24/1 -> SigSpec_24/1
  In Bus Element23/1 -> RateTs_24/1
  SigSpec_25/1 -> Out Bus Element24/1
  RateTs_25/1 -> SigSpec_25/1
  In Bus Element24/1 -> RateTs_25/1
  SigSpec_26/1 -> Out Bus Element25/1
  RateTs_26/1 -> SigSpec_26/1
  In Bus Element25/1 -> RateTs_26/1
  SigSpec_27/1 -> Out Bus Element26/1
  RateTs_27/1 -> SigSpec_27/1
  In Bus Element26/1 -> RateTs_27/1
  SigSpec_28/1 -> Out Bus Element27/1
  RateTs_28/1 -> SigSpec_28/1
  In Bus Element27/1 -> RateTs_28/1
  SigSpec_29/1 -> Out Bus Element28/1
  RateTs_29/1 -> SigSpec_29/1
  In Bus Element28/1 -> RateTs_29/1
  SigSpec_30/1 -> Out Bus Element29/1
  RateTs_30/1 -> SigSpec_30/1
  In Bus Element29/1 -> RateTs_30/1
  SigSpec_31/1 -> Out Bus Element30/1
  RateTs_31/1 -> SigSpec_31/1
  In Bus Element30/1 -> RateTs_31/1
  SigSpec_32/1 -> Out Bus Element31/1
  RateTs_32/1 -> SigSpec_32/1
  In Bus Element31/1 -> RateTs_32/1
  SigSpec_33/1 -> Out Bus Element32/1
  RateTs_33/1 -> SigSpec_33/1
  In Bus Element32/1 -> RateTs_33/1
  SigSpec_34/1 -> Out Bus Element33/1
  RateTs_34/1 -> SigSpec_34/1
  In Bus Element33/1 -> RateTs_34/1
  SigSpec_35/1 -> Out Bus Element34/1
  RateTs_35/1 -> SigSpec_35/1
  In Bus Element34/1 -> RateTs_35/1
  SigSpec_36/1 -> Out Bus Element35/1
  RateTs_36/1 -> SigSpec_36/1
  In Bus Element35/1 -> RateTs_36/1

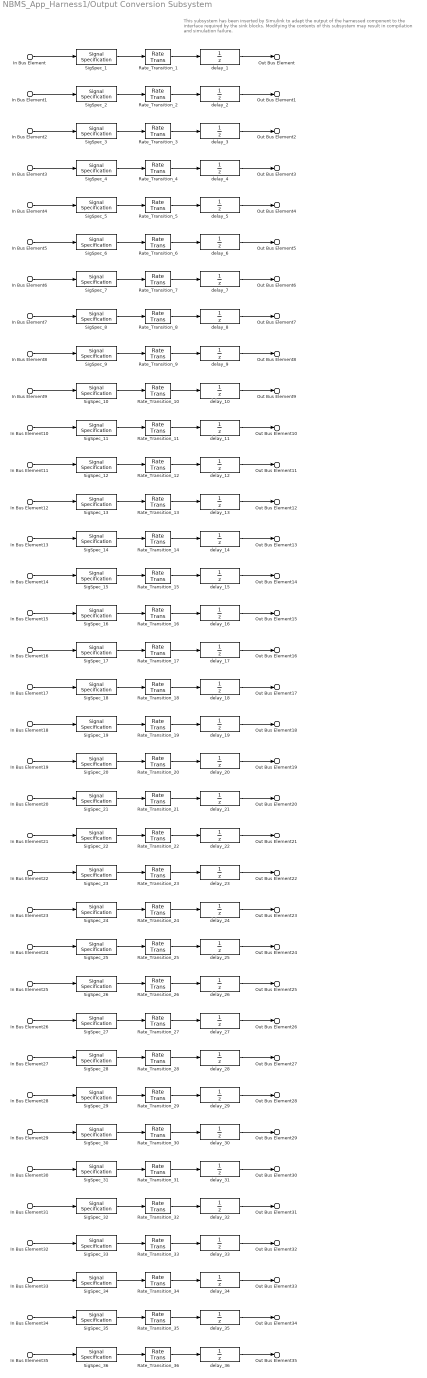
== system NBMS_App_Harness1/Output Conversion Subsystem ==
  note: This subsystem has been inserted by Simulink to adapt the output of the harnessed component to the interface required by the sink blocks.
      |  Modifying the contents of this subsystem may result in compilation and simulation failure.
  In Bus Element : Inport  PortName=Inport_1
  In Bus Element1 : Inport  Port=2  PortName=Inport_2
  In Bus Element2 : Inport  Port=3  PortName=Inport_3
  In Bus Element3 : Inport  Port=4  PortName=Inport_4
  In Bus Element4 : Inport  Port=5  PortName=Inport_5
  In Bus Element5 : Inport  Port=6  PortName=Inport_6
  In Bus Element6 : Inport  Port=7  PortName=Inport_7
  In Bus Element7 : Inport  Port=8  PortName=Inport_8
  In Bus Element8 : Inport  Port=9  PortName=Inport_9
  In Bus Element9 : Inport  Port=10  PortName=Inport_10
  In Bus Element10 : Inport  Port=11  PortName=Inport_11
  In Bus Element11 : Inport  Port=12  PortName=Inport_12
  In Bus Element12 : Inport  Port=13  PortName=Inport_13
  In Bus Element13 : Inport  Port=14  PortName=Inport_14
  In Bus Element14 : Inport  Port=15  PortName=Inport_15
  In Bus Element15 : Inport  Port=16  PortName=Inport_16
  In Bus Element16 : Inport  Port=17  PortName=Inport_17
  In Bus Element17 : Inport  Port=18  PortName=Inport_18
  In Bus Element18 : Inport  Port=19  PortName=Inport_19
  In Bus Element19 : Inport  Port=20  PortName=Inport_20
  In Bus Element20 : Inport  Port=21  PortName=Inport_21
  In Bus Element21 : Inport  Port=22  PortName=Inport_22
  In Bus Element22 : Inport  Port=23  PortName=Inport_23
  In Bus Element23 : Inport  Port=24  PortName=Inport_24
  In Bus Element24 : Inport  Port=25  PortName=Inport_25
  In Bus Element25 : Inport  Port=26  PortName=Inport_26
  In Bus Element26 : Inport  Port=27  PortName=Inport_27
  In Bus Element27 : Inport  Port=28  PortName=Inport_28
  In Bus Element28 : Inport  Port=29  PortName=Inport_29
  In Bus Element29 : Inport  Port=30  PortName=Inport_30
  In Bus Element30 : Inport  Port=31  PortName=Inport_31
  In Bus Element31 : Inport  Port=32  PortName=Inport_32
  In Bus Element32 : Inport  Port=33  PortName=Inport_33
  In Bus Element33 : Inport  Port=34  PortName=Inport_34
  In Bus Element34 : Inport  Port=35  PortName=Inport_35
  In Bus Element35 : Inport  Port=36  PortName=Inport_36
  Rate_Transition_1 : RateTransition  InitialCondition=BMS_MODE_E.BMS_SLEEP  OutPortSampleTimeOpt=Inherit
  Rate_Transition_{2..4,8..10,12..30,32..34} (28 alike) : RateTransition  OutPortSampleTimeOpt=Inherit
  Rate_Transition_11 : RateTransition  InitialCondition=Charger_Mode_Req_E.Disabled  OutPortSampleTimeOpt=Inherit
  Rate_Transition_31 : RateTransition  InitialCondition=BMS_NM_Msg_E.SLEEP  OutPortSampleTimeOpt=Inherit
  Rate_Transition_35 : RateTransition  InitialCondition=BMS_BattTempDerate_E.Temp_NoDerating  OutPortSampleTimeOpt=Inherit
  Rate_Transition_36 : RateTransition  InitialCondition=BMS_BattSoCDerate_E.SOC_NoDerating  OutPortSampleTimeOpt=Inherit
  Rate_Transition_5 : RateTransition  InitialCondition=BMS_PMosfet_STS_E.PDISCONNECTED  OutPortSampleTimeOpt=Inherit
  Rate_Transition_6 : RateTransition  InitialCondition=BMS_HVMosfet_STS_E.HV_DISCONNECTED  OutPortSampleTimeOpt=Inherit
  Rate_Transition_7 : RateTransition  InitialCondition=BMS_DCDCMosfet_STS_E.DCDC_DISCONNECTED  OutPortSampleTimeOpt=Inherit
  SigSpec_1 : SignalSpecification  OutDataTypeStr=Enum: BMS_MODE_E  Dimensions=[1]  SampleTime=0.1
  SigSpec_{2..4,8..10,16..18,32,34} (11 alike) : SignalSpecification  OutDataTypeStr=boolean  Dimensions=[1]  SampleTime=0.1
  SigSpec_11 : SignalSpecification  OutDataTypeStr=Enum: Charger_Mode_Req_E  Dimensions=[1]  SampleTime=0.1
  SigSpec_{12..13,15,19..22,25..28,30} (12 alike) : SignalSpecification  OutDataTypeStr=double  Dimensions=[1]  SampleTime=0.1
  SigSpec_14 : SignalSpecification  OutDataTypeStr=uint8  Dimensions=[1]  SampleTime=0.1
  SigSpec_23 : SignalSpecification  OutDataTypeStr=fixdt('ufix16_Sp01')  Dimensions=[1]  SampleTime=0.1
  SigSpec_24 : SignalSpecification  OutDataTypeStr=fixdt('ufix16_Sp01')  Dimensions=[1]  SampleTime=0.1
  SigSpec_29 : SignalSpecification  OutDataTypeStr=double  Dimensions=[1, 1]  SampleTime=0.1
  SigSpec_31 : SignalSpecification  OutDataTypeStr=Enum: BMS_NM_Msg_E  Dimensions=[1]  SampleTime=0.1
  SigSpec_33 : SignalSpecification  OutDataTypeStr=double  Dimensions=[1, 1]  SampleTime=0.1
  SigSpec_35 : SignalSpecification  OutDataTypeStr=Enum: BMS_BattTempDerate_E  Dimensions=[1, 1]  SampleTime=0.1
  SigSpec_36 : SignalSpecification  OutDataTypeStr=Enum: BMS_BattSoCDerate_E  Dimensions=[1]  SampleTime=0.1
  SigSpec_5 : SignalSpecification  OutDataTypeStr=Enum: BMS_PMosfet_STS_E  Dimensions=[1]  SampleTime=0.1
  SigSpec_6 : SignalSpecification  OutDataTypeStr=Enum: BMS_HVMosfet_STS_E  Dimensions=[1]  SampleTime=0.1
  SigSpec_7 : SignalSpecification  OutDataTypeStr=Enum: BMS_DCDCMosfet_STS_E  Dimensions=[1]  SampleTime=0.1
  delay_1 : UnitDelay  InitialCondition=BMS_MODE_E.BMS_SLEEP  SampleTime=-1
  delay_{2..4,8..10,12..30,32..34} (28 alike) : UnitDelay  SampleTime=-1
  delay_11 : UnitDelay  InitialCondition=Charger_Mode_Req_E.Disabled  SampleTime=-1
  delay_31 : UnitDelay  InitialCondition=BMS_NM_Msg_E.SLEEP  SampleTime=-1
  delay_35 : UnitDelay  InitialCondition=BMS_BattTempDerate_E.Temp_NoDerating  SampleTime=-1
  delay_36 : UnitDelay  InitialCondition=BMS_BattSoCDerate_E.SOC_NoDerating  SampleTime=-1
  delay_5 : UnitDelay  InitialCondition=BMS_PMosfet_STS_E.PDISCONNECTED  SampleTime=-1
  delay_6 : UnitDelay  InitialCondition=BMS_HVMosfet_STS_E.HV_DISCONNECTED  SampleTime=-1
  delay_7 : UnitDelay  InitialCondition=BMS_DCDCMosfet_STS_E.DCDC_DISCONNECTED  SampleTime=-1
  Out Bus Element : Outport  PortName=Outport_1
  Out Bus Element1 : Outport  Port=2  PortName=Outport_2
  Out Bus Element2 : Outport  Port=3  PortName=Outport_3
  Out Bus Element3 : Outport  Port=4  PortName=Outport_4
  Out Bus Element4 : Outport  Port=5  PortName=Outport_5
  Out Bus Element5 : Outport  Port=6  PortName=Outport_6
  Out Bus Element6 : Outport  Port=7  PortName=Outport_7
  Out Bus Element7 : Outport  Port=8  PortName=Outport_8
  Out Bus Element8 : Outport  Port=9  PortName=Outport_9
  Out Bus Element9 : Outport  Port=10  PortName=Outport_10
  Out Bus Element10 : Outport  Port=11  PortName=Outport_11
  Out Bus Element11 : Outport  Port=12  PortName=Outport_12
  Out Bus Element12 : Outport  Port=13  PortName=Outport_13
  Out Bus Element13 : Outport  Port=14  PortName=Outport_14
  Out Bus Element14 : Outport  Port=15  PortName=Outport_15
  Out Bus Element15 : Outport  Port=16  PortName=Outport_16
  Out Bus Element16 : Outport  Port=17  PortName=Outport_17
  Out Bus Element17 : Outport  Port=18  PortName=Outport_18
  Out Bus Element18 : Outport  Port=19  PortName=Outport_19
  Out Bus Element19 : Outport  Port=20  PortName=Outport_20
  Out Bus Element20 : Outport  Port=21  PortName=Outport_21
  Out Bus Element21 : Outport  Port=22  PortName=Outport_22
  Out Bus Element22 : Outport  Port=23  PortName=Outport_23
  Out Bus Element23 : Outport  Port=24  PortName=Outport_24
  Out Bus Element24 : Outport  Port=25  PortName=Outport_25
  Out Bus Element25 : Outport  Port=26  PortName=Outport_26
  Out Bus Element26 : Outport  Port=27  PortName=Outport_27
  Out Bus Element27 : Outport  Port=28  PortName=Outport_28
  Out Bus Element28 : Outport  Port=29  PortName=Outport_29
  Out Bus Element29 : Outport  Port=30  PortName=Outport_30
  Out Bus Element30 : Outport  Port=31  PortName=Outport_31
  Out Bus Element31 : Outport  Port=32  PortName=Outport_32
  Out Bus Element32 : Outport  Port=33  PortName=Outport_33
  Out Bus Element33 : Outport  Port=34  PortName=Outport_34
  Out Bus Element34 : Outport  Port=35  PortName=Outport_35
  Out Bus Element35 : Outport  Port=36  PortName=Outport_36
  wires:
  In Bus Element/1 -> SigSpec_1/1
  SigSpec_1/1 -> Rate_Transition_1/1
  Rate_Transition_1/1 -> delay_1/1
  delay_1/1 -> Out Bus Element/1
  In Bus Element1/1 -> SigSpec_2/1
  SigSpec_2/1 -> Rate_Transition_2/1
  Rate_Transition_2/1 -> delay_2/1
  delay_2/1 -> Out Bus Element1/1
  In Bus Element2/1 -> SigSpec_3/1
  SigSpec_3/1 -> Rate_Transition_3/1
  Rate_Transition_3/1 -> delay_3/1
  delay_3/1 -> Out Bus Element2/1
  In Bus Element3/1 -> SigSpec_4/1
  SigSpec_4/1 -> Rate_Transition_4/1
  Rate_Transition_4/1 -> delay_4/1
  delay_4/1 -> Out Bus Element3/1
  In Bus Element4/1 -> SigSpec_5/1
  SigSpec_5/1 -> Rate_Transition_5/1
  Rate_Transition_5/1 -> delay_5/1
  delay_5/1 -> Out Bus Element4/1
  In Bus Element5/1 -> SigSpec_6/1
  SigSpec_6/1 -> Rate_Transition_6/1
  Rate_Transition_6/1 -> delay_6/1
  delay_6/1 -> Out Bus Element5/1
  In Bus Element6/1 -> SigSpec_7/1
  SigSpec_7/1 -> Rate_Transition_7/1
  Rate_Transition_7/1 -> delay_7/1
  delay_7/1 -> Out Bus Element6/1
  In Bus Element7/1 -> SigSpec_8/1
  SigSpec_8/1 -> Rate_Transition_8/1
  Rate_Transition_8/1 -> delay_8/1
  delay_8/1 -> Out Bus Element7/1
  In Bus Element8/1 -> SigSpec_9/1
  SigSpec_9/1 -> Rate_Transition_9/1
  Rate_Transition_9/1 -> delay_9/1
  delay_9/1 -> Out Bus Element8/1
  In Bus Element9/1 -> SigSpec_10/1
  SigSpec_10/1 -> Rate_Transition_10/1
  Rate_Transition_10/1 -> delay_10/1
  delay_10/1 -> Out Bus Element9/1
  In Bus Element10/1 -> SigSpec_11/1
  SigSpec_11/1 -> Rate_Transition_11/1
  Rate_Transition_11/1 -> delay_11/1
  delay_11/1 -> Out Bus Element10/1
  In Bus Element11/1 -> SigSpec_12/1
  SigSpec_12/1 -> Rate_Transition_12/1
  Rate_Transition_12/1 -> delay_12/1
  delay_12/1 -> Out Bus Element11/1
  In Bus Element12/1 -> SigSpec_13/1
  SigSpec_13/1 -> Rate_Transition_13/1
  Rate_Transition_13/1 -> delay_13/1
  delay_13/1 -> Out Bus Element12/1
  In Bus Element13/1 -> SigSpec_14/1
  SigSpec_14/1 -> Rate_Transition_14/1
  Rate_Transition_14/1 -> delay_14/1
  delay_14/1 -> Out Bus Element13/1
  In Bus Element14/1 -> SigSpec_15/1
  SigSpec_15/1 -> Rate_Transition_15/1
  Rate_Transition_15/1 -> delay_15/1
  delay_15/1 -> Out Bus Element14/1
  In Bus Element15/1 -> SigSpec_16/1
  SigSpec_16/1 -> Rate_Transition_16/1
  Rate_Transition_16/1 -> delay_16/1
  delay_16/1 -> Out Bus Element15/1
  In Bus Element16/1 -> SigSpec_17/1
  SigSpec_17/1 -> Rate_Transition_17/1
  Rate_Transition_17/1 -> delay_17/1
  delay_17/1 -> Out Bus Element16/1
  In Bus Element17/1 -> SigSpec_18/1
  SigSpec_18/1 -> Rate_Transition_18/1
  Rate_Transition_18/1 -> delay_18/1
  delay_18/1 -> Out Bus Element17/1
  In Bus Element18/1 -> SigSpec_19/1
  SigSpec_19/1 -> Rate_Transition_19/1
  Rate_Transition_19/1 -> delay_19/1
  delay_19/1 -> Out Bus Element18/1
  In Bus Element19/1 -> SigSpec_20/1
  SigSpec_20/1 -> Rate_Transition_20/1
  Rate_Transition_20/1 -> delay_20/1
  delay_20/1 -> Out Bus Element19/1
  In Bus Element20/1 -> SigSpec_21/1
  SigSpec_21/1 -> Rate_Transition_21/1
  Rate_Transition_21/1 -> delay_21/1
  delay_21/1 -> Out Bus Element20/1
  In Bus Element21/1 -> SigSpec_22/1
  SigSpec_22/1 -> Rate_Transition_22/1
  Rate_Transition_22/1 -> delay_22/1
  delay_22/1 -> Out Bus Element21/1
  In Bus Element22/1 -> SigSpec_23/1
  SigSpec_23/1 -> Rate_Transition_23/1
  Rate_Transition_23/1 -> delay_23/1
  delay_23/1 -> Out Bus Element22/1
  In Bus Element23/1 -> SigSpec_24/1
  SigSpec_24/1 -> Rate_Transition_24/1
  Rate_Transition_24/1 -> delay_24/1
  delay_24/1 -> Out Bus Element23/1
  In Bus Element24/1 -> SigSpec_25/1
  SigSpec_25/1 -> Rate_Transition_25/1
  Rate_Transition_25/1 -> delay_25/1
  delay_25/1 -> Out Bus Element24/1
  In Bus Element25/1 -> SigSpec_26/1
  SigSpec_26/1 -> Rate_Transition_26/1
  Rate_Transition_26/1 -> delay_26/1
  delay_26/1 -> Out Bus Element25/1
  In Bus Element26/1 -> SigSpec_27/1
  SigSpec_27/1 -> Rate_Transition_27/1
  Rate_Transition_27/1 -> delay_27/1
  delay_27/1 -> Out Bus Element26/1
  In Bus Element27/1 -> SigSpec_28/1
  SigSpec_28/1 -> Rate_Transition_28/1
  Rate_Transition_28/1 -> delay_28/1
  delay_28/1 -> Out Bus Element27/1
  In Bus Element28/1 -> SigSpec_29/1
  SigSpec_29/1 -> Rate_Transition_29/1
  Rate_Transition_29/1 -> delay_29/1
  delay_29/1 -> Out Bus Element28/1
  In Bus Element29/1 -> SigSpec_30/1
  SigSpec_30/1 -> Rate_Transition_30/1
  Rate_Transition_30/1 -> delay_30/1
  delay_30/1 -> Out Bus Element29/1
  In Bus Element30/1 -> SigSpec_31/1
  SigSpec_31/1 -> Rate_Transition_31/1
  Rate_Transition_31/1 -> delay_31/1
  delay_31/1 -> Out Bus Element30/1
  In Bus Element31/1 -> SigSpec_32/1
  SigSpec_32/1 -> Rate_Transition_32/1
  Rate_Transition_32/1 -> delay_32/1
  delay_32/1 -> Out Bus Element31/1
  In Bus Element32/1 -> SigSpec_33/1
  SigSpec_33/1 -> Rate_Transition_33/1
  Rate_Transition_33/1 -> delay_33/1
  delay_33/1 -> Out Bus Element32/1
  In Bus Element33/1 -> SigSpec_34/1
  SigSpec_34/1 -> Rate_Transition_34/1
  Rate_Transition_34/1 -> delay_34/1
  delay_34/1 -> Out Bus Element33/1
  In Bus Element34/1 -> SigSpec_35/1
  SigSpec_35/1 -> Rate_Transition_35/1
  Rate_Transition_35/1 -> delay_35/1
  delay_35/1 -> Out Bus Element34/1
  In Bus Element35/1 -> SigSpec_36/1
  SigSpec_36/1 -> Rate_Transition_36/1
  Rate_Transition_36/1 -> delay_36/1
  delay_36/1 -> Out Bus Element35/1
